simulink library "Generator_Lib"  (R2025a)
settings: Solver=ode45  StartTime=0.0  StopTime=10.0  RelTol=1e-3  EnableMultiTasking=on
undefined symbols (not defined in the file or in its folder): DiscIntNeverNeededParam, K, Lambda, radps2rpm, tau, WT_Params, x0
libraries: fl_lib x24, nesl_utility x16, ee_lib x14, simulink x1
(part 2 of 2)

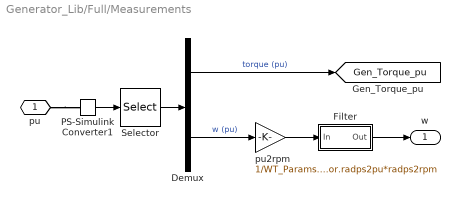
== system Generator_Lib/Full/Measurements ==
  Demux : Demux  Outputs=2
  Filter : Subsystem  mask(First-order lag supporting vector signals){b=WT_Params.Generator.generator_time_constant, x_initial=0}
      mask prompts: b "Filter time constant"; x_initial "Initial output"
      mask help: Models a lag of the form 1/(b*s+1) where s is the Laplace operator.
  PS-Simulink Converter1 : nesl_utility/PS-Simulink Converter  PhysicalDomain=network_engine_domain  SubClassName=ps_output  LeftPortType=input  RightPortType=output  PseudoPeriodic=off  Frequencies=[]  VectorFormat=inherit  Unit=inherit  AffineConversion=off
  Selector : Selector  InputPortWidth=8  IndexOptions=Index vector (dialog)  Indices=[1 2]  OutputSizes=1
  pu2rpm : Gain  Gain=1/WT_Params.Generator.radps2pu*radps2rpm
  pu : PMIOPort  Side=Left
  w : Outport
  tag scope: Gen_Torque_pu=global
  wires:
  pu2rpm/1 -> Filter/1(In)
  Demux/1 -> [Gen_Torque_pu]  "torque (pu)"
  Demux/2 -> pu2rpm/1  "w (pu)"
  Selector/1 -> Demux/1
  PS-Simulink Converter1/1 -> Selector/1
  Filter/1(Out) -> w/1
  connections:
  pu/RConn1 -- PS-Simulink Converter1/LConn1

== system Generator_Lib/Grid/Mutual RL Pos-Zero (SI) ==
  Coupled : ee_lib/Passive/Lines/Coupled Lines (Three-Phase)  port_option=ee.enum.threePhasePort.composite  prm=1  La=1e-3 H  Lb=1e-3 H  Lc=1e-3 H  L=Ls_si H  Lmab=3e-4 H  Lmac=3e-4 H  Lmbc=3e-4 H  Lm=Lm_si H  Ra=0.001 Ohm  Rb=0.001 Ohm  Rc=0.001 Ohm  R=Rs_si Ohm  Rmab=0 Ohm  Rmac=0 Ohm  Rmbc=0 Ohm  Rm=Rm_si Ohm  Ga=1e-9 1/Ohm  Gb=1e-9 1/Ohm  Gc=1e-9 1/Ohm  G=0 1/Ohm  I_L_specify=off  I_L_priority=High  I_L=[0, 0, 0] A  I_L_nominal_specify=off  I_L_nominal_value=1  I_L_nominal_unit=A  i_La_specify=off  i_La_priority=High  i_La=0 A  i_La_nominal_specify=off  i_La_nominal_value=1  i_La_nominal_unit=A  i_Lb_specify=off  i_Lb_priority=High  i_Lb=0 A  i_Lb_nominal_specify=off  i_Lb_nominal_value=1  i_Lb_nominal_unit=A  i_Lc_specify=off  i_Lc_priority=High  i_Lc=0 A  i_Lc_nominal_specify=off  i_Lc_nominal_value=1  i_Lc_nominal_unit=A
      settings: InternalSimscapePortConfiguration="{\"Bottom\":[],\"Left\":[{\"id\":\"N1\",\"label\":\"~1\",\"type\":\"foundation.electrical.three_phase\"}],\"Right\":[{\"id\":\"N2\",\"label\":\"~2\",\"type\":\"foundation.electrical.three_phase\"}],\"Top\":[]}"
  ~1 : PMIOPort  Side=Left
  ~2 : PMIOPort  Port=2  Side=Right
  connections:
  Coupled/LConn1 -- ~1/RConn1
  Coupled/RConn1 -- ~2/RConn1

== system Generator_Lib/Grid/Pi-Section Pos-Zero (SI) ==
  Electrical Reference : fl_lib/Electrical/Electrical Elements/Electrical Reference
  Electrical Reference1 : fl_lib/Electrical/Electrical Elements/Electrical Reference
  line : ee_lib/Passive/Lines/Transmission Line (Three-Phase)  length=length km  freq=Fnom Hz  R=Rs_si Ohm/km  L=Ls_si mH/m  M=Lm_si mH/m  Cl=Cl_si mF/m  Cg=Cg_si mF/m  Rm=Rm_si Ohm/km  ModelTwoSections=ee.enum.enable.no  N=1  InterfacePosition=0.5 km  N1sec=1  N2sec=1  Access_ground=ee.enum.enable.no  R_parasitic=1e-6 Ohm  G_parasitic=1e-6 1/Ohm
      settings: InternalSimscapePortConfiguration="{\"Bottom\":[],\"Left\":[{\"id\":\"N1\",\"label\":\"~1\",\"type\":\"foundation.electrical.three_phase\"},{\"id\":\"g1\",\"label\":\"g1\",\"type\":\"foundation.electrical.electrical\"}],\"Right\":[{\"id\":\"N2\",\"label\":\"~2\",\"type\":\"foundation.electrical.three_phase\"},{\"id\":\"g2\",\"label\":\"g2\",\"type\":\"foundation.electrical.electrical\"}],\"Top\":[]}"
  ~1 : PMIOPort  Side=Left
  ~2 : PMIOPort  Port=2  Side=Right
  connections:
  line/RConn2 -- Electrical Reference1/LConn1
  line/LConn2 -- Electrical Reference/LConn1
  line/RConn1 -- ~2/RConn1
  line/LConn1 -- ~1/RConn1

== system Generator_Lib/Simple/Actuator Dynamics ==
  In : Inport
  Gain : Gain  Gain=1/b
  Integrator : Integrator  InitialCondition=x_initial
  Sum : Sum  Inputs=|+-  InputSameDT=on  SaturateOnIntegerOverflow=on  OutDataTypeStr=Inherit: Same as first input
  Out : Outport  VectorParamsAs1DForOutWhenUnconnected=off
  wires:
  Gain/1 -> Out/1, Sum/2
  Integrator/1 -> Gain/1
  In/1 -> Sum/1
  Sum/1 -> Integrator/1

== system Generator_Lib/Simple/Speed Sensor ==
  Ideal Rotational Motion Sensor : fl_lib/Mechanical/Mechanical Sensors/Ideal Rotational Motion Sensor  reference=foundation.enum.MeasurementReference.difference  acceleration_port=false  velocity_port=true  position_port=true  wrap_angle=simscape.enum.onoff.off  offset=0 rad
  Mechanical Rotational Reference1 : fl_lib/Mechanical/Rotational Elements/Mechanical Rotational Reference
  PS-Simulink Converter : nesl_utility/PS-Simulink Converter  PhysicalDomain=network_engine_domain  SubClassName=ps_output  LeftPortType=input  RightPortType=output  PseudoPeriodic=off  Frequencies=[]  VectorFormat=1-D array  Unit=1  AffineConversion=off
  R : PMIOPort  Side=Left
  S : Outport  VectorParamsAs1DForOutWhenUnconnected=off
  wires:
  PS-Simulink Converter/1 -> S/1
  connections:
  Ideal Rotational Motion Sensor/RConn2 -- PS-Simulink Converter/LConn1
  R/RConn1 -- Ideal Rotational Motion Sensor/LConn1
  Mechanical Rotational Reference1/LConn1 -- Ideal Rotational Motion Sensor/RConn1

== system Generator_Lib/Simple/Torque Sensor ==
  Ideal Torque Sensor : fl_lib/Mechanical/Mechanical Sensors/Ideal Torque Sensor
  PS-Simulink Converter : nesl_utility/PS-Simulink Converter  PhysicalDomain=network_engine_domain  SubClassName=ps_output  LeftPortType=input  RightPortType=output  PseudoPeriodic=off  Frequencies=[]  VectorFormat=1-D array  Unit=1  AffineConversion=off
  radps2rpm1 : Gain  Gain=1/500
  R : PMIOPort  Side=Left
  C : PMIOPort  Port=2  Side=Right
  tag scope: Gen_Torque_pu=global
  wires:
  radps2rpm1/1 -> [Gen_Torque_pu]  "Electromagnetic torque Te (pu)"
  PS-Simulink Converter/1 -> radps2rpm1/1
  connections:
  PS-Simulink Converter/LConn1 -- Ideal Torque Sensor/RConn2
  C/RConn1 -- Ideal Torque Sensor/RConn1
  R/RConn1 -- Ideal Torque Sensor/LConn1

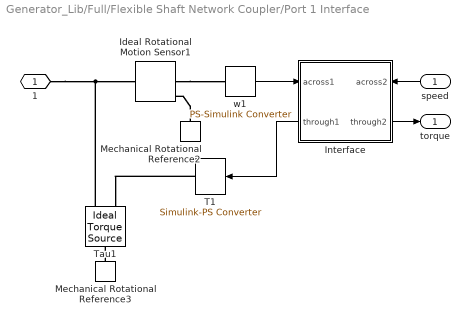
== system Generator_Lib/Full/Flexible Shaft Network Coupler/Port 1 Interface ==
  speed : Inport
  Ideal Rotational Motion Sensor1 : fl_lib/Mechanical/Mechanical Sensors/Ideal Rotational Motion Sensor  reference=foundation.enum.MeasurementReference.difference  acceleration_port=false  velocity_port=true  position_port=true  wrap_angle=simscape.enum.onoff.off  offset=0 rad
  Interface : Subsystem  Variant=on  VariantControlMode=label  VariantControl=Variant1  LabelModeActiveChoice=Continuous
      settings: PortSchema="{\"entries\":[{\"content\":{\"sides\":[{\"content\":{\"connectorIds\":[\"In1\",\"Out2\"]},\"type\":\"ConnectorPlacement.EquallySpacedRectSide\",\"uuid\":\"aa56821c-7799-44e3-b228-553c5b43a68d\"},{\"content\":{\"connectorIds\":[\"In2\",\"Out1\"],\"side\":\"RIGHT\"},\"type\":\"ConnectorPlacement.EquallySpacedRectSide\",\"uuid\":\"8658dee5-55e2-4f33-bdec-e6600ce27fc1\"},{\"content\":{\"connectorIds\":[],\"side\":\"TOP\"},\"type\":\"ConnectorPlacement.EquallySpacedRectSide\",\"uuid\":\"2effe9c6-8e61-4f0c-a39b-329d9ffc707d\"}]},\"type\":\"ConnectorPlacement.EquallySpacedConnector\",\"uuid\":\"c8fc8444-dfc7-49a5-9550-b957635f7d8f\"}],\"packageUris\":[\"http://schema.mathworks.com/mf0/Connector/R2020b\"],\"version\":\"1.0\"}"
  Mechanical Rotational Reference2 : fl_lib/Mechanical/Rotational Elements/Mechanical Rotational Reference
  Mechanical Rotational Reference3 : fl_lib/Mechanical/Rotational Elements/Mechanical Rotational Reference
  T1 : nesl_utility/Simulink-PS Converter  PhysicalDomain=network_engine_domain  SubClassName=ps_input  LeftPortType=input  RightPortType=output  PseudoPeriodic=off  Frequencies=[]  NoiseDistribution=none  NoiseParameters=[]  Unit=N*m  AffineConversion=off  FilteringAndDerivatives=zero  SimscapeFilterOrder=1  InputFilterTimeConstant=0.001  UdotUserProvided=1
  Tau1 : fl_lib/Mechanical/Mechanical Sources/Ideal Torque Source
  w1 : nesl_utility/PS-Simulink Converter  PhysicalDomain=network_engine_domain  SubClassName=ps_output  LeftPortType=input  RightPortType=output  PseudoPeriodic=off  Frequencies=[]  VectorFormat=1-D array  Unit=rad/s  AffineConversion=off
  1 : PMIOPort  Side=Left
  torque : Outport
  wires:
  speed/1 -> Interface/2(across2)
  Interface/2(through1) -> T1/1
  w1/1 -> Interface/1(across1)
  Interface/1(through2) -> torque/1
  connections:
  1/RConn1 -- Ideal Rotational Motion Sensor1/LConn1 -- Tau1/RConn2
  Mechanical Rotational Reference2/LConn1 -- Ideal Rotational Motion Sensor1/RConn1
  Ideal Rotational Motion Sensor1/RConn2 -- w1/LConn1
  Mechanical Rotational Reference3/LConn1 -- Tau1/LConn1
  T1/RConn1 -- Tau1/RConn1

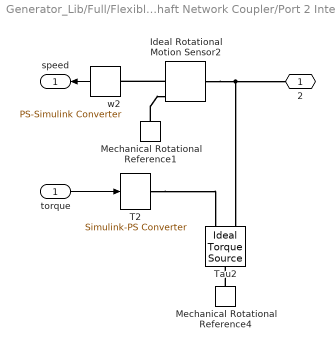
== system Generator_Lib/Full/Flexible Shaft Network Coupler/Port 2 Interface ==
  torque : Inport
  Ideal Rotational Motion Sensor2 : fl_lib/Mechanical/Mechanical Sensors/Ideal Rotational Motion Sensor  reference=foundation.enum.MeasurementReference.difference  acceleration_port=false  velocity_port=true  position_port=true  wrap_angle=simscape.enum.onoff.off  offset=0 rad
  Mechanical Rotational Reference1 : fl_lib/Mechanical/Rotational Elements/Mechanical Rotational Reference
  Mechanical Rotational Reference4 : fl_lib/Mechanical/Rotational Elements/Mechanical Rotational Reference
  T2 : nesl_utility/Simulink-PS Converter  PhysicalDomain=network_engine_domain  SubClassName=ps_input  LeftPortType=input  RightPortType=output  PseudoPeriodic=off  Frequencies=[]  NoiseDistribution=none  NoiseParameters=[]  Unit=N*m  AffineConversion=off  FilteringAndDerivatives=zero  SimscapeFilterOrder=1  InputFilterTimeConstant=0.001  UdotUserProvided=1
  Tau2 : fl_lib/Mechanical/Mechanical Sources/Ideal Torque Source
  w2 : nesl_utility/PS-Simulink Converter  PhysicalDomain=network_engine_domain  SubClassName=ps_output  LeftPortType=input  RightPortType=output  PseudoPeriodic=off  Frequencies=[]  VectorFormat=1-D array  Unit=rad/s  AffineConversion=off
  2 : PMIOPort  Side=Right
  speed : Outport
  wires:
  torque/1 -> T2/1
  w2/1 -> speed/1
  connections:
  T2/RConn1 -- Tau2/RConn1
  Mechanical Rotational Reference1/LConn1 -- Ideal Rotational Motion Sensor2/RConn1
  Ideal Rotational Motion Sensor2/RConn2 -- w2/LConn1
  Ideal Rotational Motion Sensor2/LConn1 -- 2/RConn1 -- Tau2/RConn2
  Mechanical Rotational Reference4/LConn1 -- Tau2/LConn1

== system Generator_Lib/Full/Measurements/Filter ==
  In : Inport
  Gain : Gain  Gain=1/b
  Integrator : Integrator  InitialCondition=x_initial
  Sum : Sum  Inputs=|+-  InputSameDT=on  SaturateOnIntegerOverflow=on  OutDataTypeStr=Inherit: Same as first input
  Out : Outport  VectorParamsAs1DForOutWhenUnconnected=off
  wires:
  Gain/1 -> Out/1, Sum/2
  Integrator/1 -> Gain/1
  In/1 -> Sum/1
  Sum/1 -> Integrator/1

== system Generator_Lib/Full/Flexible Shaft Network Coupler/Port 1 Interface/Interface ==
  across1 : Inport
  across2 : Inport  Port=2
  Continuous : Subsystem  VariantControl=Continuous
  Discrete : Subsystem  VariantControl=Discrete
  through2 : Outport
  through1 : Outport  Port=2

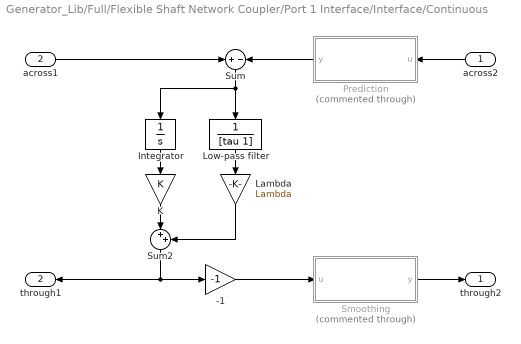
== system Generator_Lib/Full/Flexible Shaft Network Coupler/Port 1 Interface/Interface/Continuous ==
  across2 : Inport
  across1 : Inport  Port=2
  -1 : Gain  Gain=-1  SaturateOnIntegerOverflow=on  OutDataTypeStr=Inherit: Same as input  ParamDataTypeStr=Inherit: Same as input
  Integrator : Integrator  InitialCondition=x0
  K : Gain  Gain=K  SaturateOnIntegerOverflow=on  OutDataTypeStr=Inherit: Same as input  ParamDataTypeStr=Inherit: Same as input
  Lambda : Gain  Gain=Lambda  SaturateOnIntegerOverflow=on  OutDataTypeStr=Inherit: Same as input  ParamDataTypeStr=Inherit: Same as input
  Low-pass filter : TransferFcn  Numerator=1  Denominator=[tau 1]
  Prediction : Subsystem  Commented=through  mask(Prediction (discrete->continuous)){h2=h2}
      mask prompts: h2 "physmod:simscape:couplers:SimscapeNetworkCouplersLib:PortUDiscreteSampleTimes_MP"
      mask help: physmod:simscape:couplers:SimscapeNetworkCouplersLib:Predictiondiscretecontinuous_MD
      mask DialogControl h2 Prompt: Port u discrete sample time (s)
  Smoothing : Subsystem  Commented=through  mask(Smoothing (continuous->discrete)){tsSmoothing=tsSmoothing, smoothing0=-through0}
      mask prompts: tsSmoothing "physmod:simscape:couplers:SimscapeNetworkCouplersLib:SmoothingTimeConstants_MP"; smoothing0 "physmod:simscape:couplers:SimscapeNetworkCouplersLib:InitialOutput_MP"
      mask help: physmod:simscape:couplers:SimscapeNetworkCouplersLib:Smoothingcontinuousdiscrete_MD
      mask DialogControl tsSmoothing Prompt: Smoothing time constant (s)
      mask DialogControl smoothing0 Prompt: Initial output
  Sum : Sum  Inputs=+-  InputSameDT=on  SaturateOnIntegerOverflow=on  OutDataTypeStr=Inherit: Same as first input
  Sum2 : Sum  Inputs=|++
  through2 : Outport
  through1 : Outport  Port=2
  wires:
  K/1 -> Sum2/1
  Sum2/1 -> through1/1, -1/1
  across2/1 -> Prediction/1(u)
  Low-pass filter/1 -> Lambda/1
  Integrator/1 -> K/1
  Sum/1 -> Integrator/1, Low-pass filter/1
  across1/1 -> Sum/1
  Lambda/1 -> Sum2/2
  Prediction/1(y) -> Sum/2
  Smoothing/1(y) -> through2/1
  -1/1 -> Smoothing/1(u)

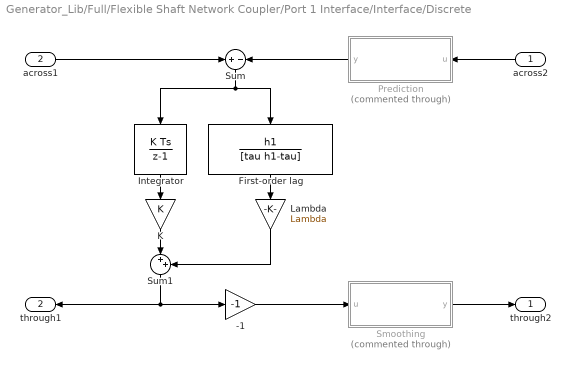
== system Generator_Lib/Full/Flexible Shaft Network Coupler/Port 1 Interface/Interface/Discrete ==
  across2 : Inport
  across1 : Inport  Port=2
  -1 : Gain  Gain=-1  SaturateOnIntegerOverflow=on  OutDataTypeStr=Inherit: Same as input  ParamDataTypeStr=Inherit: Same as input
  First-order lag : DiscreteTransferFcn  Numerator=h1  Denominator=[tau h1-tau]  SampleTime=h1
  Integrator : DiscreteIntegrator  InitialCondition=x0  SampleTime=h1  ICPrevOutput=DiscIntNeverNeededParam  ICPrevScaledInput=DiscIntNeverNeededParam
  K : Gain  Gain=K  SaturateOnIntegerOverflow=on  OutDataTypeStr=Inherit: Same as input  ParamDataTypeStr=Inherit: Same as input
  Lambda : Gain  Gain=Lambda  SaturateOnIntegerOverflow=on  OutDataTypeStr=Inherit: Same as input  ParamDataTypeStr=Inherit: Same as input
  Prediction : Subsystem  Commented=through  mask(Prediction (slow->fast)){h2=h2, h1=h1}
      mask prompts: h2 "physmod:simscape:couplers:SimscapeNetworkCouplersLib:PortUDiscreteSampleTimes_MP"; h1 "physmod:simscape:couplers:SimscapeNetworkCouplersLib:PortYDiscreteSampleTimes_MP"
      mask help: physmod:simscape:couplers:SimscapeNetworkCouplersLib:Predictionslowfast_MD
      mask DialogControl h2 Prompt: Port u discrete sample time (s)
      mask DialogControl h1 Prompt: Port y discrete sample time (s)
  Smoothing : Subsystem  Commented=through  mask(Smoothing (fast->slow)){nSmooth=nSmooth, h1=h1, smoothing0=-through0}
      mask prompts: nSmooth "physmod:simscape:couplers:SimscapeNetworkCouplersLib:NumberOfSamplesOverWhichToSmooth_MP"; h1 "physmod:simscape:couplers:SimscapeNetworkCouplersLib:PortUDiscreteSampleTimes_MP"; smoothing0 "physmod:simscape:couplers:SimscapeNetworkCouplersLib:InitialOutput_MP"
      mask help: physmod:simscape:couplers:SimscapeNetworkCouplersLib:Smoothingfastslow_MD
      mask DialogControl nSmooth Prompt: Number of samples over which to smooth
      mask DialogControl h1 Prompt: Port u discrete sample time (s)
      mask DialogControl smoothing0 Prompt: Initial output
  Sum : Sum  Inputs=+-  InputSameDT=on  SaturateOnIntegerOverflow=on  OutDataTypeStr=Inherit: Same as first input
  Sum1 : Sum  Inputs=|++
  through2 : Outport
  through1 : Outport  Port=2
  wires:
  First-order lag/1 -> Lambda/1
  Integrator/1 -> K/1
  K/1 -> Sum1/1
  across1/1 -> Sum/1
  Sum/1 -> Integrator/1, First-order lag/1
  across2/1 -> Prediction/1(u)
  Sum1/1 -> through1/1, -1/1
  Lambda/1 -> Sum1/2
  Prediction/1(y) -> Sum/2
  Smoothing/1(y) -> through2/1
  -1/1 -> Smoothing/1(u)

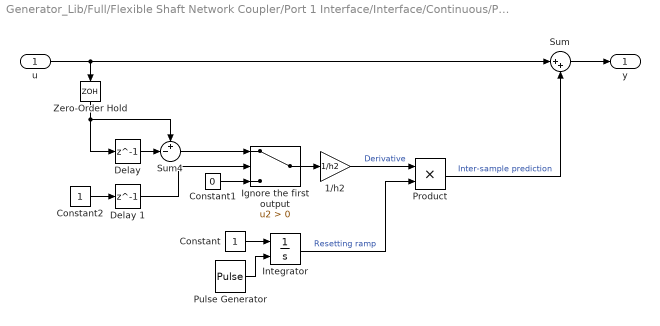
== system Generator_Lib/Full/Flexible Shaft Network Coupler/Port 1 Interface/Interface/Continuous/Prediction ==
  u : Inport
  1/h2 : Gain  Gain=1/h2
  Constant : Constant  SampleTime=h2
  Constant1 : Constant  Value=0  SampleTime=h2
  Constant2 : Constant  SampleTime=h2
  "Delay " : Delay  DelayLength=1  SampleTime=h2
  Delay 1 : Delay  DelayLength=1  SampleTime=h2
  Ignore the first output : Switch  Criteria=u2 > Threshold  SaturateOnIntegerOverflow=off  InputSameDT=off
  Integrator : Integrator  ExternalReset=either  LimitOutput=on  UpperSaturationLimit=1  LowerSaturationLimit=0
  Product : Product
  Pulse Generator : DiscretePulseGenerator  SampleTime=h2
  Sum : Sum  Inputs=|++
  Sum4 : Sum  Inputs=+-|
  Zero-Order Hold : ZeroOrderHold  SampleTime=h2
  y : Outport
  wires:
  Product/1 -> Sum/2  "Inter-sample prediction"
  Zero-Order Hold/1 -> Sum4/1, "Delay "/1
  u/1 -> Sum/1, Zero-Order Hold/1
  "Delay "/1 -> Sum4/2
  1/h2/1 -> Product/1  "Derivative"
  Sum/1 -> y/1
  Integrator/1 -> Product/2  "Resetting ramp"
  Constant/1 -> Integrator/1
  Pulse Generator/1 -> Integrator/2
  Ignore the first output/1 -> 1/h2/1
  Sum4/1 -> Ignore the first output/1
  Constant1/1 -> Ignore the first output/3
  Delay 1/1 -> Ignore the first output/2
  Constant2/1 -> Delay 1/1

== system Generator_Lib/Full/Flexible Shaft Network Coupler/Port 1 Interface/Interface/Continuous/Smoothing ==
  u : Inport
  Gain : Gain  Gain=1/tsSmoothing
  Integrator : Integrator  InitialCondition=smoothing0
  Sum : Sum  Inputs=|+-
  y : Outport
  wires:
  u/1 -> Sum/1
  Integrator/1 -> Sum/2, y/1
  Gain/1 -> Integrator/1
  Sum/1 -> Gain/1

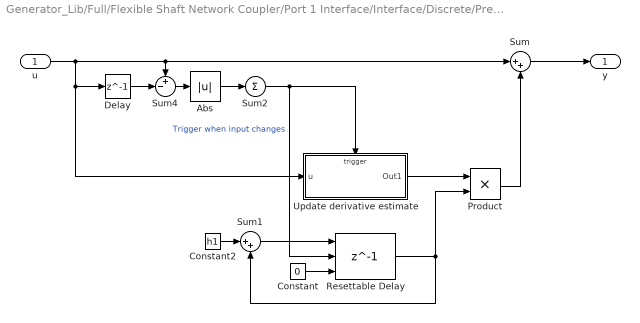
== system Generator_Lib/Full/Flexible Shaft Network Coupler/Port 1 Interface/Interface/Discrete/Prediction ==
  u : Inport
  Abs : Abs  SaturateOnIntegerOverflow=off
  Constant : Constant  Value=0  SampleTime=h1
  Constant2 : Constant  Value=h1  SampleTime=h1
  "Delay " : Delay  DelayLength=1  SampleTime=h1
  Product : Product
  Resettable Delay : Delay  DelayLength=1  InitialConditionSource=Input port  ExternalReset=Rising  SampleTime=h1
      settings: InputPortMap=u0,r5,p4
  Sum : Sum  Inputs=|++
  Sum1 : Sum  Inputs=|++
  Sum2 : Sum  Inputs=+
  Sum4 : Sum  Inputs=+-|
  Update derivative estimate : Subsystem  TreatAsAtomicUnit=on
  y : Outport
  wires:
  Abs/1 -> Sum2/1
  Sum2/1 -> Resettable Delay/2, Update derivative estimate/Trigger  "Trigger when input changes"
  Sum1/1 -> Resettable Delay/1
  Sum/1 -> y/1
  "Delay "/1 -> Sum4/2
  Product/1 -> Sum/2
  Update derivative estimate/1(Out1) -> Product/1
  u/1 -> Update derivative estimate/1(u), "Delay "/1, Sum/1, Sum4/1
  Sum4/1 -> Abs/1
  Resettable Delay/1 -> Product/2, Sum1/2
  Constant2/1 -> Sum1/1
  Constant/1 -> Resettable Delay/3

== system Generator_Lib/Full/Flexible Shaft Network Coupler/Port 1 Interface/Interface/Discrete/Smoothing ==
  u : Inport
  Gain : Gain  Gain=1/nSmooth
  Sum of Elements : Sum  Inputs=+
  Tapped Delay : simulink/Discrete/Tapped Delay  vinit=smoothing0  samptime=h1  NumDelays=nSmooth  DelayOrder=Oldest  includeCurrent=off
  y : Outport
  wires:
  Gain/1 -> y/1
  Sum of Elements/1 -> Gain/1
  Tapped Delay/1 -> Sum of Elements/1
  u/1 -> Tapped Delay/1

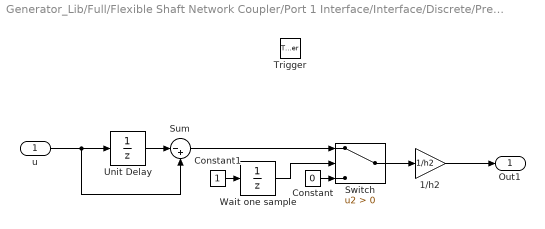
== system Generator_Lib/Full/Flexible Shaft Network Coupler/Port 1 Interface/Interface/Discrete/Prediction/Update derivative estimate ==
  u : Inport
  Trigger : TriggerPort  VariantControl=(inherit)
  1/h2 : Gain  Gain=1/h2
  Constant : Constant  Value=0  SampleTime=-1
  Constant1 : Constant  SampleTime=-1
  Sum : Sum  Inputs=|-+
  Switch : Switch  Criteria=u2 > Threshold  SaturateOnIntegerOverflow=off  InputSameDT=off
  Unit Delay : UnitDelay  SampleTime=-1  HasFrameUpgradeWarning=on
  Wait one sample : UnitDelay  SampleTime=-1  HasFrameUpgradeWarning=on
  Out1 : Outport
  wires:
  Unit Delay/1 -> Sum/1
  u/1 -> Unit Delay/1, Sum/2
  1/h2/1 -> Out1/1
  Switch/1 -> 1/h2/1
  Sum/1 -> Switch/1
  Constant/1 -> Switch/3
  Wait one sample/1 -> Switch/2
  Constant1/1 -> Wait one sample/1
